simulink model "strainBasedMotorDrive_v3"  (Simulink 7.9)
settings: Solver=FixedStepDiscrete  SolverMode=SingleTasking  StartTime=0.0  StopTime=inf  FixedStep=1.25e-7  RelTol=1e-3
libraries: dsPICdrivers x5
settings Model: Creator=ij8977  LastModifiedBy=ij8977  ExtModeTrigDuration=10000
settings SolverCC: PositivePriorityOrder=on
settings OptimizationCC: OptimizeModelRefInitCode=on  LifeSpan=Inf
settings DebuggingCC: FcnCallInpInsideContextMsg=Use local settings  StrictBusMsg=Warning
settings RTWCC: SystemTargetFile=pic32.tlc  MakeCommand=make_CreateMPLAB  TemplateMakefile=pic32_gcc.tmf  PostCodeGenCommand=dsPIC_Compile()  Description=Embedded Target for Microchip dsPIC (real-time)  ProcessScript=pic32_make_rtw_hook
settings CodeAppCC: IgnoreCustomStorageClasses=off
settings STFCustomTargetCC: CodeReplacementLibrary=ANSI_C  IncludeMdlTerminateFcn=off  CombineOutputUpdateFcns=on  SuppressErrorStatus=on  ERTCustomFileBanners=on  SupportContinuousTime=off  SupportNonInlinedSFcns=off  GRTInterface=off  SystemTargetFile=pic32.tlc
settings ERTTargetCC: CodeReplacementLibrary=ANSI_C  MultiwordLength=2048  ParMdlRefBuildCompliant=off  CompOptLevelCompliant=off  ConcurrentExecutionCompliant=off  IncludeMdlTerminateFcn=off  SuppressErrorStatus=on  ERTFirstTimeCompliant=off  ModelStepFunctionPrototypeControlCompliant=off  CPPClassGenCompliant=off  ExtModeMexFile=noextcomm  InlinedParameterPlacement=NonHierarchical  ERTSrcFileBannerTemplate=dsPIC_code_template.cgt  ERTHdrFileBannerTemplate=dsPIC_code_template.cgt  ERTDataSrcFileTemplate=dsPIC_code_template.cgt  ERTDataHdrFileTemplate=dsPIC_code_template.cgt  ERTCustomFileTemplate=dsPIC_main.tlc  ConvertIfToSwitch=off  SuppressUnreachableDefaultCases=off
settings CustomProperty: DataType=string  Value=C:\PROGRA~1\MATLAB\R2012a\bin\win32\gmake

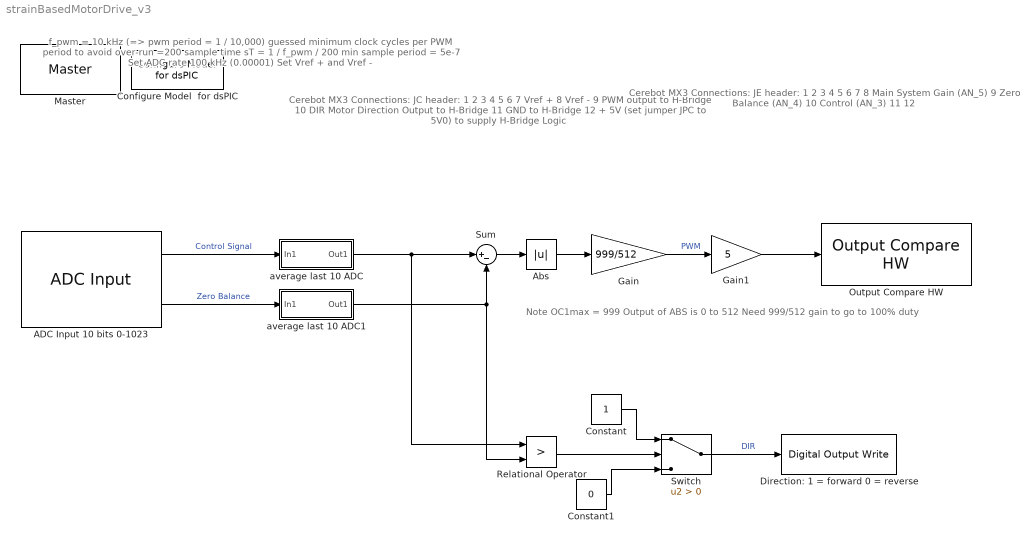
== system strainBasedMotorDrive_v3 ==
  note: f_pwm = 10 kHz
      | (=> pwm period = 1 / 10,000)
      | guessed minimum clock cycles per
      | PWM period to avoid over-run =200
      | sample time sT = 1  /  f_pwm / 200
      | min sample period = 5e-7
      |
      | Set ADC rate 100 kHz (0.00001)
      |
      | Set Vref + and Vref -
  note: Cerebot MX3 Connections:
      | JC header:
      | 1
      | 2
      | 3
      | 4
      | 5
      | 6
      | 7   Vref +
      | 8   Vref -
      | 9   PWM output to H-Bridge
      | 10 DIR Motor Direction Output to H-Bridge
      | 11 GND to H-Bridge
      | 12 + 5V (set jumper JPC to 5V0) to supply H-Bridge Logic
  note: Note OC1max = 999
      | Output of ABS is 0 to 512
      | Need 999/512 gain to go to 100% duty
  note: Cerebot MX3 Connections:
      | JE header:
      | 1
      | 2
      | 3
      | 4
      | 5
      | 6
      | 7
      | 8     Main System Gain (AN_5)
      | 9     Zero Balance (AN_4)
      | 10   Control (AN_3)
      | 11
      | 12
  ADC Input 10 bits 0-1023 : dsPICdrivers/Peripheral I//O/ADC Input  Tag=dsPIC_ADC  Priority=5  ADC_TYPE=10 bits  ADC_MODE=Continuous sampling & get last channel value  NbrSampleStep=10  VoltRefpopup="AVdd  -  AVss"  OutFormatBitspopup=0000 00dd dddd dddd : Integer  InterruptPriority=6  ANCHANNELS=[3 4]  MaxName=ANmax = 1023  Rin=2e2  ADCS=12  SAMC=1  Temperature=25  DMAChannel=0  SampleTime=.00001  Status="OK  |  Tsmp=1.625e-07 |  T/Channel=2.113e-06 |  Tall=4.225e-05"  SSRC=Timer3 (OC_HW PWM)
  Abs : Abs  OutDataTypeStr=uint16
  Configure Model  for dsPIC : dsPICdrivers/Simulink Configuration/Configure Model  for dsPIC
  Constant : Constant  OutDataTypeStr=boolean
  Constant1 : Constant  Value=0  OutDataTypeStr=boolean
  Direction: 1 = forward 0 = reverse : dsPICdrivers/Digital I//O/Digital Output Write  Tag=dsPIC_Digital_Output  Priority=5  PORT=D  Pin=[1]  Simultaneous=off  OrderingInOutPopup=None
  Gain : Gain  Gain=999/512  OutDataTypeStr=uint16
  Gain1 : Gain  Gain=5  OutDataTypeStr=uint16
  Master : dsPICdrivers/Master  Tag=dsPIC_MASTER  Priority=1  TimeStepType=Timer1  picType=32MX320F128H  fcy=40000000  Quartz_33f=8e6  PLLActive_33f=on  fcyDesired_33f=40e6  tmr1="[1  4  0]"  tmr1Info="Time Step : 1.25e-07  ;   Error : 0%  PR1=4"  tmr2345="[0  1  0  0]"  tmr2345cfg=[-1 -1 -1 -1]  IOautoConf=on  typePort="[ 0   0   0   0   0   0   0   0   0   0   0   0   0   0   0   0   0   0   0   8   8   0   0   0   0   0   0   0   0   0   0   0   0   0   0   0   0   0   0   0   0   0   0   0   0   0   0   0  24  10   0   0   0   0   0   0   0   0   0   0   0   0   0   0   0   0   0   0   0   0   0   0   0   0   0   0   0   0   0   0   0   0   0   0   0   0   0   0   0   0   0   0   0   0   0   0   0   0   0   0   0   0   0   0   0   0   0   0   0   0   0   0 ]"  TRIS="[ 65535  65535  65535  65532  65535  65535  65535 ]"  ADPCFG=0  MasterBusyPort=None  MasterOverloadPort=None  FOSC=Quartz (XT - HS)  ClockSwitchMonitor=Both disabled  TempProtection_33f=TEMP_ON  FPBOR=<empty>  PWRT=disable  MCLR=<empty>  ICD=ICS_PGD1  JTAGEN=JTAGEN_OFF  PowerSave=off  OverrideFcy=off  NewFcy=1e6  PR2345="[65535   3999  65535  65535]"
  Output Compare HW : dsPICdrivers/Peripheral I//O/Output Compare HW  Tag=dsPIC_OC_HW_out  Priority=5  OC_Mode=PWM duty cycle (robust)  Timer=3  CHANNEL=[1]  Channel_UP_Down_Periode=[5]  PeriodeInput=off  MaxChannel=0.0001  MaxName=' OCmax '  Precision=[11.9658]  Status=OK  SafeMarge=[0]  PortLetter=[68]  PortNumber=[0]  MaxValues=[3999]  NPORTS=1
  Relational Operator : RelationalOperator  Operator=>  OutDataTypeStr=boolean
  Sum : Sum  Inputs=|+-  OutDataTypeStr=int16
  Switch : Switch  Criteria=u2 > Threshold  OutDataTypeStr=Inherit: Inherit via back propagation  ZeroCross=off
  average last 10 ADC : Subsystem
  average last 10 ADC1 : Subsystem
  wires:
  Switch/1 -> Direction: 1 = forward 0 = reverse/1  "DIR"
  Constant1/1 -> Switch/3
  Constant/1 -> Switch/1
  Relational Operator/1 -> Switch/2
  ADC Input 10 bits 0-1023/1 -> average last 10 ADC/1(In1)  "Control Signal"
  Sum/1 -> Abs/1
  Abs/1 -> Gain/1
  Gain/1 -> Gain1/1  "PWM"
  ADC Input 10 bits 0-1023/2 -> average last 10 ADC1/1(In1)  "Zero Balance"
  average last 10 ADC1/1(Out1) -> Sum/2, Relational Operator/2
  average last 10 ADC/1(Out1) -> Sum/1, Relational Operator/1
  Gain1/1 -> Output Compare HW/1

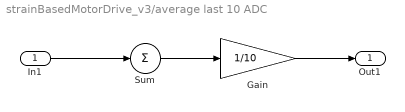
== system strainBasedMotorDrive_v3/average last 10 ADC ==
  In1 : Inport
  Gain : Gain  Gain=1/10  OutDataTypeStr=uint16
  Sum : Sum  Inputs=+  AccumDataTypeStr=uint16
  Out1 : Outport
  wires:
  Gain/1 -> Out1/1
  In1/1 -> Sum/1
  Sum/1 -> Gain/1

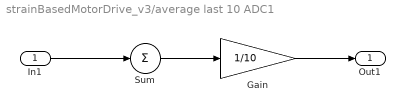
== system strainBasedMotorDrive_v3/average last 10 ADC1 ==
  In1 : Inport
  Gain : Gain  Gain=1/10  OutDataTypeStr=uint16
  Sum : Sum  Inputs=+  AccumDataTypeStr=uint16
  Out1 : Outport
  wires:
  Sum/1 -> Gain/1
  In1/1 -> Sum/1
  Gain/1 -> Out1/1
